simulink library "lib_LargeBuildingModel"  (R2026a)
settings: Solver=VariableStepAuto
libraries: WallSelector_lib x380, ExternalWall_lib x188, RoomWithAirVolume x140, fl_lib x139, RoomLevelControl_lib x1
(part 11 of 12)

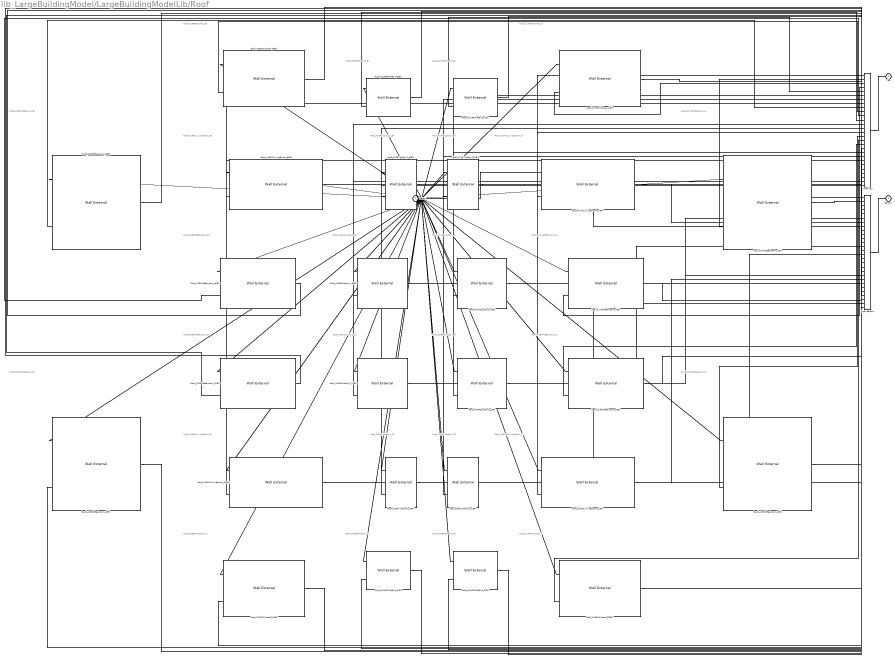
== system lib_LargeBuildingModel/LargeBuildingModelLib/Roof ==
  note: Roof_A17R1(LivingRoom_A)
  note: Roof_A17R2(Bedroom_A)
  note: Roof_A17R3(Kitchen_A)
  note: Roof_A17R4(Bathroom_A)
  note: Roof_A17R5(FireExit_A)
  note: Roof_A17R6(Lobby1_A)
  note: Roof_A17R7(Lobby2_A)
  note: Roof_A18R1(LivingRoom_B)
  note: Roof_A18R2(Bedroom_B)
  note: Roof_A18R3(Kitchen_B)
  note: Roof_A18R4(Bathroom_B)
  note: Roof_A18R5(FireExit_B)
  note: Roof_A18R6(Lobby1_B)
  note: Roof_A18R7(Lobby2_B)
  note: Roof_A19R1(LivingRoom_C)
  note: Roof_A19R2(Bedroom_C)
  note: Roof_A19R3(Kitchen_C)
  note: Roof_A19R4(Bathroom_C)
  note: Roof_A19R5(FireExit_C)
  note: Roof_A19R6(Lobby1_C)
  note: Roof_A19R7(Lobby2_C)
  note: Roof_A20R1(LivingRoom_D)
  note: Roof_A20R2(Bedroom_D)
  note: Roof_A20R3(Kitchen_D)
  note: Roof_A20R4(Bathroom_D)
  note: Roof_A20R5(FireExit_D)
  note: Roof_A20R6(Lobby1_D)
  note: Roof_A20R7(Lobby2_D)
  ArrayBottom : SimscapeArrayConnection  Domain=foundation.thermal.thermal  ConcatenateDimension=1  NumScalarElements=28
  ArrayTop : SimscapeArrayConnection  Domain=foundation.thermal.thermal  ConcatenateDimension=1  NumScalarElements=28
  Roof_A17R1(LivingRoom_A)Blk : ExternalWall_lib/Wall External  extWallModel=wallExternalModelOption.wallSolar  wallLength=2.4384 % Parameterized on : 13-Jun-2026 10:47:16 m  wallHeight=4.572 % Parameterized on : 13-Jun-2026 10:47:16 m  wallThickness=0.03 % Parameterized on : 13-Jun-2026 10:47:16 m  wallMaterialDen=1400 % Parameterized on : 13-Jun-2026 10:47:30 kg/m^3  wallMaterialCp=1000 % Parameterized on : 13-Jun-2026 10:47:30 J/(K*kg)  wallAbsorptivity=0.5  wallThermalK=0.7 % Parameterized on : 13-Jun-2026 10:47:30 W/(K*m)  winLength=1 m  winHeight=0.5 m  winThickness=0.007 m  winMaterialDen=2500 kg/m^3  winMaterialCp=787 J/(K*kg)  winAbsorptivity=0.35  winThermalK=1 W/(K*m)  winTransmissivity=0.45  ventLength=0.1 m  ventHeight=0.1 m  extToWallHTC=30 % Parameterized on : 13-Jun-2026 10:47:30 W/(K*m^2)  intToRoomHTC=30 % Parameterized on : 13-Jun-2026 10:47:30 W/(K*m^2)  iniT=300 % Parameterized on : 13-Jun-2026 10:47:30 K  latitude=5  longitude=5  localTime=5  dayLightS=0  surfAngle=90 deg  surfUnitV=[0, -1]  startYear=2025  startMonth=1  startDay=1  startHr=1  numHrsData=24  interp_method=simscape.enum.interpolation.linear  extrap_method=simscape.enum.extrapolation.nearest
  Roof_A17R2(Bedroom_A)Blk : ExternalWall_lib/Wall External  extWallModel=wallExternalModelOption.wallSolar  wallLength=4.2672 % Parameterized on : 13-Jun-2026 10:47:16 m  wallHeight=4.572 % Parameterized on : 13-Jun-2026 10:47:16 m  wallThickness=0.03 % Parameterized on : 13-Jun-2026 10:47:16 m  wallMaterialDen=1400 % Parameterized on : 13-Jun-2026 10:47:30 kg/m^3  wallMaterialCp=1000 % Parameterized on : 13-Jun-2026 10:47:30 J/(K*kg)  wallAbsorptivity=0.5  wallThermalK=0.7 % Parameterized on : 13-Jun-2026 10:47:30 W/(K*m)  winLength=1 m  winHeight=0.5 m  winThickness=0.007 m  winMaterialDen=2500 kg/m^3  winMaterialCp=787 J/(K*kg)  winAbsorptivity=0.35  winThermalK=1 W/(K*m)  winTransmissivity=0.45  ventLength=0.1 m  ventHeight=0.1 m  extToWallHTC=30 % Parameterized on : 13-Jun-2026 10:47:30 W/(K*m^2)  intToRoomHTC=30 % Parameterized on : 13-Jun-2026 10:47:30 W/(K*m^2)  iniT=300 % Parameterized on : 13-Jun-2026 10:47:30 K  latitude=5  longitude=5  localTime=5  dayLightS=0  surfAngle=90 deg  surfUnitV=[0, -1]  startYear=2025  startMonth=1  startDay=1  startHr=1  numHrsData=24  interp_method=simscape.enum.interpolation.linear  extrap_method=simscape.enum.extrapolation.nearest
  Roof_A17R3(Kitchen_A)Blk : ExternalWall_lib/Wall External  extWallModel=wallExternalModelOption.wallSolar  wallLength=2.7432 % Parameterized on : 13-Jun-2026 10:47:16 m  wallHeight=3.9624 % Parameterized on : 13-Jun-2026 10:47:16 m  wallThickness=0.03 % Parameterized on : 13-Jun-2026 10:47:16 m  wallMaterialDen=1400 % Parameterized on : 13-Jun-2026 10:47:30 kg/m^3  wallMaterialCp=1000 % Parameterized on : 13-Jun-2026 10:47:30 J/(K*kg)  wallAbsorptivity=0.5  wallThermalK=0.7 % Parameterized on : 13-Jun-2026 10:47:30 W/(K*m)  winLength=1 m  winHeight=0.5 m  winThickness=0.007 m  winMaterialDen=2500 kg/m^3  winMaterialCp=787 J/(K*kg)  winAbsorptivity=0.35  winThermalK=1 W/(K*m)  winTransmissivity=0.45  ventLength=0.1 m  ventHeight=0.1 m  extToWallHTC=30 % Parameterized on : 13-Jun-2026 10:47:30 W/(K*m^2)  intToRoomHTC=30 % Parameterized on : 13-Jun-2026 10:47:30 W/(K*m^2)  iniT=300 % Parameterized on : 13-Jun-2026 10:47:30 K  latitude=5  longitude=5  localTime=5  dayLightS=0  surfAngle=90 deg  surfUnitV=[0, -1]  startYear=2025  startMonth=1  startDay=1  startHr=1  numHrsData=24  interp_method=simscape.enum.interpolation.linear  extrap_method=simscape.enum.extrapolation.nearest
  Roof_A17R4(Bathroom_A)Blk : ExternalWall_lib/Wall External  extWallModel=wallExternalModelOption.wallSolar  wallLength=2.4384 % Parameterized on : 13-Jun-2026 10:47:16 m  wallHeight=3.6576 % Parameterized on : 13-Jun-2026 10:47:16 m  wallThickness=0.03 % Parameterized on : 13-Jun-2026 10:47:16 m  wallMaterialDen=1400 % Parameterized on : 13-Jun-2026 10:47:30 kg/m^3  wallMaterialCp=1000 % Parameterized on : 13-Jun-2026 10:47:30 J/(K*kg)  wallAbsorptivity=0.5  wallThermalK=0.7 % Parameterized on : 13-Jun-2026 10:47:30 W/(K*m)  winLength=1 m  winHeight=0.5 m  winThickness=0.007 m  winMaterialDen=2500 kg/m^3  winMaterialCp=787 J/(K*kg)  winAbsorptivity=0.35  winThermalK=1 W/(K*m)  winTransmissivity=0.45  ventLength=0.1 m  ventHeight=0.1 m  extToWallHTC=30 % Parameterized on : 13-Jun-2026 10:47:30 W/(K*m^2)  intToRoomHTC=30 % Parameterized on : 13-Jun-2026 10:47:30 W/(K*m^2)  iniT=300 % Parameterized on : 13-Jun-2026 10:47:30 K  latitude=5  longitude=5  localTime=5  dayLightS=0  surfAngle=90 deg  surfUnitV=[0, -1]  startYear=2025  startMonth=1  startDay=1  startHr=1  numHrsData=24  interp_method=simscape.enum.interpolation.linear  extrap_method=simscape.enum.extrapolation.nearest
  Roof_A17R5(FireExit_A)Blk : ExternalWall_lib/Wall External  extWallModel=wallExternalModelOption.wallSolar  wallLength=1.8288 % Parameterized on : 13-Jun-2026 10:47:16 m  wallHeight=2.1336 % Parameterized on : 13-Jun-2026 10:47:16 m  wallThickness=0.03 % Parameterized on : 13-Jun-2026 10:47:16 m  wallMaterialDen=1400 % Parameterized on : 13-Jun-2026 10:47:30 kg/m^3  wallMaterialCp=1000 % Parameterized on : 13-Jun-2026 10:47:30 J/(K*kg)  wallAbsorptivity=0.5  wallThermalK=0.7 % Parameterized on : 13-Jun-2026 10:47:30 W/(K*m)  winLength=1 m  winHeight=0.5 m  winThickness=0.007 m  winMaterialDen=2500 kg/m^3  winMaterialCp=787 J/(K*kg)  winAbsorptivity=0.35  winThermalK=1 W/(K*m)  winTransmissivity=0.45  ventLength=0.1 m  ventHeight=0.1 m  extToWallHTC=30 % Parameterized on : 13-Jun-2026 10:47:30 W/(K*m^2)  intToRoomHTC=30 % Parameterized on : 13-Jun-2026 10:47:30 W/(K*m^2)  iniT=300 % Parameterized on : 13-Jun-2026 10:47:30 K  latitude=5  longitude=5  localTime=5  dayLightS=0  surfAngle=90 deg  surfUnitV=[0, -1]  startYear=2025  startMonth=1  startDay=1  startHr=1  numHrsData=24  interp_method=simscape.enum.interpolation.linear  extrap_method=simscape.enum.extrapolation.nearest
  Roof_A17R6(Lobby1_A)Blk : ExternalWall_lib/Wall External  extWallModel=wallExternalModelOption.wallSolar  wallLength=2.4384 % Parameterized on : 13-Jun-2026 10:47:16 m  wallHeight=2.4384 % Parameterized on : 13-Jun-2026 10:47:16 m  wallThickness=0.03 % Parameterized on : 13-Jun-2026 10:47:16 m  wallMaterialDen=1400 % Parameterized on : 13-Jun-2026 10:47:30 kg/m^3  wallMaterialCp=1000 % Parameterized on : 13-Jun-2026 10:47:30 J/(K*kg)  wallAbsorptivity=0.5  wallThermalK=0.7 % Parameterized on : 13-Jun-2026 10:47:30 W/(K*m)  winLength=1 m  winHeight=0.5 m  winThickness=0.007 m  winMaterialDen=2500 kg/m^3  winMaterialCp=787 J/(K*kg)  winAbsorptivity=0.35  winThermalK=1 W/(K*m)  winTransmissivity=0.45  ventLength=0.1 m  ventHeight=0.1 m  extToWallHTC=30 % Parameterized on : 13-Jun-2026 10:47:30 W/(K*m^2)  intToRoomHTC=30 % Parameterized on : 13-Jun-2026 10:47:30 W/(K*m^2)  iniT=300 % Parameterized on : 13-Jun-2026 10:47:30 K  latitude=5  longitude=5  localTime=5  dayLightS=0  surfAngle=90 deg  surfUnitV=[0, -1]  startYear=2025  startMonth=1  startDay=1  startHr=1  numHrsData=24  interp_method=simscape.enum.interpolation.linear  extrap_method=simscape.enum.extrapolation.nearest
  Roof_A17R7(Lobby2_A)Blk : ExternalWall_lib/Wall External  extWallModel=wallExternalModelOption.wallSolar  wallLength=2.4384 % Parameterized on : 13-Jun-2026 10:47:16 m  wallHeight=1.524 % Parameterized on : 13-Jun-2026 10:47:16 m  wallThickness=0.03 % Parameterized on : 13-Jun-2026 10:47:16 m  wallMaterialDen=1400 % Parameterized on : 13-Jun-2026 10:47:30 kg/m^3  wallMaterialCp=1000 % Parameterized on : 13-Jun-2026 10:47:30 J/(K*kg)  wallAbsorptivity=0.5  wallThermalK=0.7 % Parameterized on : 13-Jun-2026 10:47:30 W/(K*m)  winLength=1 m  winHeight=0.5 m  winThickness=0.007 m  winMaterialDen=2500 kg/m^3  winMaterialCp=787 J/(K*kg)  winAbsorptivity=0.35  winThermalK=1 W/(K*m)  winTransmissivity=0.45  ventLength=0.1 m  ventHeight=0.1 m  extToWallHTC=30 % Parameterized on : 13-Jun-2026 10:47:30 W/(K*m^2)  intToRoomHTC=30 % Parameterized on : 13-Jun-2026 10:47:30 W/(K*m^2)  iniT=300 % Parameterized on : 13-Jun-2026 10:47:30 K  latitude=5  longitude=5  localTime=5  dayLightS=0  surfAngle=90 deg  surfUnitV=[0, -1]  startYear=2025  startMonth=1  startDay=1  startHr=1  numHrsData=24  interp_method=simscape.enum.interpolation.linear  extrap_method=simscape.enum.extrapolation.nearest
  Roof_A18R1(LivingRoom_B)Blk : ExternalWall_lib/Wall External  extWallModel=wallExternalModelOption.wallSolar  wallLength=2.4384 % Parameterized on : 13-Jun-2026 10:47:16 m  wallHeight=4.572 % Parameterized on : 13-Jun-2026 10:47:16 m  wallThickness=0.03 % Parameterized on : 13-Jun-2026 10:47:16 m  wallMaterialDen=1400 % Parameterized on : 13-Jun-2026 10:47:30 kg/m^3  wallMaterialCp=1000 % Parameterized on : 13-Jun-2026 10:47:30 J/(K*kg)  wallAbsorptivity=0.5  wallThermalK=0.7 % Parameterized on : 13-Jun-2026 10:47:30 W/(K*m)  winLength=1 m  winHeight=0.5 m  winThickness=0.007 m  winMaterialDen=2500 kg/m^3  winMaterialCp=787 J/(K*kg)  winAbsorptivity=0.35  winThermalK=1 W/(K*m)  winTransmissivity=0.45  ventLength=0.1 m  ventHeight=0.1 m  extToWallHTC=30 % Parameterized on : 13-Jun-2026 10:47:30 W/(K*m^2)  intToRoomHTC=30 % Parameterized on : 13-Jun-2026 10:47:30 W/(K*m^2)  iniT=300 % Parameterized on : 13-Jun-2026 10:47:30 K  latitude=5  longitude=5  localTime=5  dayLightS=0  surfAngle=90 deg  surfUnitV=[0, -1]  startYear=2025  startMonth=1  startDay=1  startHr=1  numHrsData=24  interp_method=simscape.enum.interpolation.linear  extrap_method=simscape.enum.extrapolation.nearest
  Roof_A18R2(Bedroom_B)Blk : ExternalWall_lib/Wall External  extWallModel=wallExternalModelOption.wallSolar  wallLength=4.2672 % Parameterized on : 13-Jun-2026 10:47:16 m  wallHeight=4.572 % Parameterized on : 13-Jun-2026 10:47:16 m  wallThickness=0.03 % Parameterized on : 13-Jun-2026 10:47:16 m  wallMaterialDen=1400 % Parameterized on : 13-Jun-2026 10:47:30 kg/m^3  wallMaterialCp=1000 % Parameterized on : 13-Jun-2026 10:47:31 J/(K*kg)  wallAbsorptivity=0.5  wallThermalK=0.7 % Parameterized on : 13-Jun-2026 10:47:31 W/(K*m)  winLength=1 m  winHeight=0.5 m  winThickness=0.007 m  winMaterialDen=2500 kg/m^3  winMaterialCp=787 J/(K*kg)  winAbsorptivity=0.35  winThermalK=1 W/(K*m)  winTransmissivity=0.45  ventLength=0.1 m  ventHeight=0.1 m  extToWallHTC=30 % Parameterized on : 13-Jun-2026 10:47:31 W/(K*m^2)  intToRoomHTC=30 % Parameterized on : 13-Jun-2026 10:47:31 W/(K*m^2)  iniT=300 % Parameterized on : 13-Jun-2026 10:47:31 K  latitude=5  longitude=5  localTime=5  dayLightS=0  surfAngle=90 deg  surfUnitV=[0, -1]  startYear=2025  startMonth=1  startDay=1  startHr=1  numHrsData=24  interp_method=simscape.enum.interpolation.linear  extrap_method=simscape.enum.extrapolation.nearest
  Roof_A18R3(Kitchen_B)Blk : ExternalWall_lib/Wall External  extWallModel=wallExternalModelOption.wallSolar  wallLength=2.7432 % Parameterized on : 13-Jun-2026 10:47:16 m  wallHeight=3.9624 % Parameterized on : 13-Jun-2026 10:47:16 m  wallThickness=0.03 % Parameterized on : 13-Jun-2026 10:47:16 m  wallMaterialDen=1400 % Parameterized on : 13-Jun-2026 10:47:31 kg/m^3  wallMaterialCp=1000 % Parameterized on : 13-Jun-2026 10:47:31 J/(K*kg)  wallAbsorptivity=0.5  wallThermalK=0.7 % Parameterized on : 13-Jun-2026 10:47:31 W/(K*m)  winLength=1 m  winHeight=0.5 m  winThickness=0.007 m  winMaterialDen=2500 kg/m^3  winMaterialCp=787 J/(K*kg)  winAbsorptivity=0.35  winThermalK=1 W/(K*m)  winTransmissivity=0.45  ventLength=0.1 m  ventHeight=0.1 m  extToWallHTC=30 % Parameterized on : 13-Jun-2026 10:47:31 W/(K*m^2)  intToRoomHTC=30 % Parameterized on : 13-Jun-2026 10:47:31 W/(K*m^2)  iniT=300 % Parameterized on : 13-Jun-2026 10:47:31 K  latitude=5  longitude=5  localTime=5  dayLightS=0  surfAngle=90 deg  surfUnitV=[0, -1]  startYear=2025  startMonth=1  startDay=1  startHr=1  numHrsData=24  interp_method=simscape.enum.interpolation.linear  extrap_method=simscape.enum.extrapolation.nearest
  Roof_A18R4(Bathroom_B)Blk : ExternalWall_lib/Wall External  extWallModel=wallExternalModelOption.wallSolar  wallLength=2.4384 % Parameterized on : 13-Jun-2026 10:47:16 m  wallHeight=3.6576 % Parameterized on : 13-Jun-2026 10:47:16 m  wallThickness=0.03 % Parameterized on : 13-Jun-2026 10:47:16 m  wallMaterialDen=1400 % Parameterized on : 13-Jun-2026 10:47:31 kg/m^3  wallMaterialCp=1000 % Parameterized on : 13-Jun-2026 10:47:31 J/(K*kg)  wallAbsorptivity=0.5  wallThermalK=0.7 % Parameterized on : 13-Jun-2026 10:47:31 W/(K*m)  winLength=1 m  winHeight=0.5 m  winThickness=0.007 m  winMaterialDen=2500 kg/m^3  winMaterialCp=787 J/(K*kg)  winAbsorptivity=0.35  winThermalK=1 W/(K*m)  winTransmissivity=0.45  ventLength=0.1 m  ventHeight=0.1 m  extToWallHTC=30 % Parameterized on : 13-Jun-2026 10:47:31 W/(K*m^2)  intToRoomHTC=30 % Parameterized on : 13-Jun-2026 10:47:31 W/(K*m^2)  iniT=300 % Parameterized on : 13-Jun-2026 10:47:31 K  latitude=5  longitude=5  localTime=5  dayLightS=0  surfAngle=90 deg  surfUnitV=[0, -1]  startYear=2025  startMonth=1  startDay=1  startHr=1  numHrsData=24  interp_method=simscape.enum.interpolation.linear  extrap_method=simscape.enum.extrapolation.nearest
  Roof_A18R5(FireExit_B)Blk : ExternalWall_lib/Wall External  extWallModel=wallExternalModelOption.wallSolar  wallLength=1.8288 % Parameterized on : 13-Jun-2026 10:47:16 m  wallHeight=2.1336 % Parameterized on : 13-Jun-2026 10:47:16 m  wallThickness=0.03 % Parameterized on : 13-Jun-2026 10:47:16 m  wallMaterialDen=1400 % Parameterized on : 13-Jun-2026 10:47:31 kg/m^3  wallMaterialCp=1000 % Parameterized on : 13-Jun-2026 10:47:31 J/(K*kg)  wallAbsorptivity=0.5  wallThermalK=0.7 % Parameterized on : 13-Jun-2026 10:47:31 W/(K*m)  winLength=1 m  winHeight=0.5 m  winThickness=0.007 m  winMaterialDen=2500 kg/m^3  winMaterialCp=787 J/(K*kg)  winAbsorptivity=0.35  winThermalK=1 W/(K*m)  winTransmissivity=0.45  ventLength=0.1 m  ventHeight=0.1 m  extToWallHTC=30 % Parameterized on : 13-Jun-2026 10:47:31 W/(K*m^2)  intToRoomHTC=30 % Parameterized on : 13-Jun-2026 10:47:31 W/(K*m^2)  iniT=300 % Parameterized on : 13-Jun-2026 10:47:31 K  latitude=5  longitude=5  localTime=5  dayLightS=0  surfAngle=90 deg  surfUnitV=[0, -1]  startYear=2025  startMonth=1  startDay=1  startHr=1  numHrsData=24  interp_method=simscape.enum.interpolation.linear  extrap_method=simscape.enum.extrapolation.nearest
  Roof_A18R6(Lobby1_B)Blk : ExternalWall_lib/Wall External  extWallModel=wallExternalModelOption.wallSolar  wallLength=2.4384 % Parameterized on : 13-Jun-2026 10:47:16 m  wallHeight=2.4384 % Parameterized on : 13-Jun-2026 10:47:16 m  wallThickness=0.03 % Parameterized on : 13-Jun-2026 10:47:16 m  wallMaterialDen=1400 % Parameterized on : 13-Jun-2026 10:47:31 kg/m^3  wallMaterialCp=1000 % Parameterized on : 13-Jun-2026 10:47:31 J/(K*kg)  wallAbsorptivity=0.5  wallThermalK=0.7 % Parameterized on : 13-Jun-2026 10:47:31 W/(K*m)  winLength=1 m  winHeight=0.5 m  winThickness=0.007 m  winMaterialDen=2500 kg/m^3  winMaterialCp=787 J/(K*kg)  winAbsorptivity=0.35  winThermalK=1 W/(K*m)  winTransmissivity=0.45  ventLength=0.1 m  ventHeight=0.1 m  extToWallHTC=30 % Parameterized on : 13-Jun-2026 10:47:31 W/(K*m^2)  intToRoomHTC=30 % Parameterized on : 13-Jun-2026 10:47:31 W/(K*m^2)  iniT=300 % Parameterized on : 13-Jun-2026 10:47:31 K  latitude=5  longitude=5  localTime=5  dayLightS=0  surfAngle=90 deg  surfUnitV=[0, -1]  startYear=2025  startMonth=1  startDay=1  startHr=1  numHrsData=24  interp_method=simscape.enum.interpolation.linear  extrap_method=simscape.enum.extrapolation.nearest
  Roof_A18R7(Lobby2_B)Blk : ExternalWall_lib/Wall External  extWallModel=wallExternalModelOption.wallSolar  wallLength=2.4384 % Parameterized on : 13-Jun-2026 10:47:16 m  wallHeight=1.524 % Parameterized on : 13-Jun-2026 10:47:16 m  wallThickness=0.03 % Parameterized on : 13-Jun-2026 10:47:16 m  wallMaterialDen=1400 % Parameterized on : 13-Jun-2026 10:47:31 kg/m^3  wallMaterialCp=1000 % Parameterized on : 13-Jun-2026 10:47:31 J/(K*kg)  wallAbsorptivity=0.5  wallThermalK=0.7 % Parameterized on : 13-Jun-2026 10:47:31 W/(K*m)  winLength=1 m  winHeight=0.5 m  winThickness=0.007 m  winMaterialDen=2500 kg/m^3  winMaterialCp=787 J/(K*kg)  winAbsorptivity=0.35  winThermalK=1 W/(K*m)  winTransmissivity=0.45  ventLength=0.1 m  ventHeight=0.1 m  extToWallHTC=30 % Parameterized on : 13-Jun-2026 10:47:31 W/(K*m^2)  intToRoomHTC=30 % Parameterized on : 13-Jun-2026 10:47:31 W/(K*m^2)  iniT=300 % Parameterized on : 13-Jun-2026 10:47:31 K  latitude=5  longitude=5  localTime=5  dayLightS=0  surfAngle=90 deg  surfUnitV=[0, -1]  startYear=2025  startMonth=1  startDay=1  startHr=1  numHrsData=24  interp_method=simscape.enum.interpolation.linear  extrap_method=simscape.enum.extrapolation.nearest
  Roof_A19R1(LivingRoom_C)Blk : ExternalWall_lib/Wall External  extWallModel=wallExternalModelOption.wallSolar  wallLength=2.4384 % Parameterized on : 13-Jun-2026 10:47:16 m  wallHeight=4.572 % Parameterized on : 13-Jun-2026 10:47:16 m  wallThickness=0.03 % Parameterized on : 13-Jun-2026 10:47:16 m  wallMaterialDen=1400 % Parameterized on : 13-Jun-2026 10:47:31 kg/m^3  wallMaterialCp=1000 % Parameterized on : 13-Jun-2026 10:47:31 J/(K*kg)  wallAbsorptivity=0.5  wallThermalK=0.7 % Parameterized on : 13-Jun-2026 10:47:31 W/(K*m)  winLength=1 m  winHeight=0.5 m  winThickness=0.007 m  winMaterialDen=2500 kg/m^3  winMaterialCp=787 J/(K*kg)  winAbsorptivity=0.35  winThermalK=1 W/(K*m)  winTransmissivity=0.45  ventLength=0.1 m  ventHeight=0.1 m  extToWallHTC=30 % Parameterized on : 13-Jun-2026 10:47:31 W/(K*m^2)  intToRoomHTC=30 % Parameterized on : 13-Jun-2026 10:47:31 W/(K*m^2)  iniT=300 % Parameterized on : 13-Jun-2026 10:47:31 K  latitude=5  longitude=5  localTime=5  dayLightS=0  surfAngle=90 deg  surfUnitV=[0, -1]  startYear=2025  startMonth=1  startDay=1  startHr=1  numHrsData=24  interp_method=simscape.enum.interpolation.linear  extrap_method=simscape.enum.extrapolation.nearest
  Roof_A19R2(Bedroom_C)Blk : ExternalWall_lib/Wall External  extWallModel=wallExternalModelOption.wallSolar  wallLength=4.2672 % Parameterized on : 13-Jun-2026 10:47:16 m  wallHeight=4.572 % Parameterized on : 13-Jun-2026 10:47:16 m  wallThickness=0.03 % Parameterized on : 13-Jun-2026 10:47:16 m  wallMaterialDen=1400 % Parameterized on : 13-Jun-2026 10:47:31 kg/m^3  wallMaterialCp=1000 % Parameterized on : 13-Jun-2026 10:47:31 J/(K*kg)  wallAbsorptivity=0.5  wallThermalK=0.7 % Parameterized on : 13-Jun-2026 10:47:31 W/(K*m)  winLength=1 m  winHeight=0.5 m  winThickness=0.007 m  winMaterialDen=2500 kg/m^3  winMaterialCp=787 J/(K*kg)  winAbsorptivity=0.35  winThermalK=1 W/(K*m)  winTransmissivity=0.45  ventLength=0.1 m  ventHeight=0.1 m  extToWallHTC=30 % Parameterized on : 13-Jun-2026 10:47:31 W/(K*m^2)  intToRoomHTC=30 % Parameterized on : 13-Jun-2026 10:47:31 W/(K*m^2)  iniT=300 % Parameterized on : 13-Jun-2026 10:47:31 K  latitude=5  longitude=5  localTime=5  dayLightS=0  surfAngle=90 deg  surfUnitV=[0, -1]  startYear=2025  startMonth=1  startDay=1  startHr=1  numHrsData=24  interp_method=simscape.enum.interpolation.linear  extrap_method=simscape.enum.extrapolation.nearest
  Roof_A19R3(Kitchen_C)Blk : ExternalWall_lib/Wall External  extWallModel=wallExternalModelOption.wallSolar  wallLength=2.7432 % Parameterized on : 13-Jun-2026 10:47:16 m  wallHeight=3.9624 % Parameterized on : 13-Jun-2026 10:47:16 m  wallThickness=0.03 % Parameterized on : 13-Jun-2026 10:47:16 m  wallMaterialDen=1400 % Parameterized on : 13-Jun-2026 10:47:31 kg/m^3  wallMaterialCp=1000 % Parameterized on : 13-Jun-2026 10:47:31 J/(K*kg)  wallAbsorptivity=0.5  wallThermalK=0.7 % Parameterized on : 13-Jun-2026 10:47:31 W/(K*m)  winLength=1 m  winHeight=0.5 m  winThickness=0.007 m  winMaterialDen=2500 kg/m^3  winMaterialCp=787 J/(K*kg)  winAbsorptivity=0.35  winThermalK=1 W/(K*m)  winTransmissivity=0.45  ventLength=0.1 m  ventHeight=0.1 m  extToWallHTC=30 % Parameterized on : 13-Jun-2026 10:47:31 W/(K*m^2)  intToRoomHTC=30 % Parameterized on : 13-Jun-2026 10:47:31 W/(K*m^2)  iniT=300 % Parameterized on : 13-Jun-2026 10:47:31 K  latitude=5  longitude=5  localTime=5  dayLightS=0  surfAngle=90 deg  surfUnitV=[0, -1]  startYear=2025  startMonth=1  startDay=1  startHr=1  numHrsData=24  interp_method=simscape.enum.interpolation.linear  extrap_method=simscape.enum.extrapolation.nearest
  Roof_A19R4(Bathroom_C)Blk : ExternalWall_lib/Wall External  extWallModel=wallExternalModelOption.wallSolar  wallLength=2.4384 % Parameterized on : 13-Jun-2026 10:47:16 m  wallHeight=3.6576 % Parameterized on : 13-Jun-2026 10:47:16 m  wallThickness=0.03 % Parameterized on : 13-Jun-2026 10:47:16 m  wallMaterialDen=1400 % Parameterized on : 13-Jun-2026 10:47:31 kg/m^3  wallMaterialCp=1000 % Parameterized on : 13-Jun-2026 10:47:31 J/(K*kg)  wallAbsorptivity=0.5  wallThermalK=0.7 % Parameterized on : 13-Jun-2026 10:47:31 W/(K*m)  winLength=1 m  winHeight=0.5 m  winThickness=0.007 m  winMaterialDen=2500 kg/m^3  winMaterialCp=787 J/(K*kg)  winAbsorptivity=0.35  winThermalK=1 W/(K*m)  winTransmissivity=0.45  ventLength=0.1 m  ventHeight=0.1 m  extToWallHTC=30 % Parameterized on : 13-Jun-2026 10:47:31 W/(K*m^2)  intToRoomHTC=30 % Parameterized on : 13-Jun-2026 10:47:31 W/(K*m^2)  iniT=300 % Parameterized on : 13-Jun-2026 10:47:31 K  latitude=5  longitude=5  localTime=5  dayLightS=0  surfAngle=90 deg  surfUnitV=[0, -1]  startYear=2025  startMonth=1  startDay=1  startHr=1  numHrsData=24  interp_method=simscape.enum.interpolation.linear  extrap_method=simscape.enum.extrapolation.nearest
  Roof_A19R5(FireExit_C)Blk : ExternalWall_lib/Wall External  extWallModel=wallExternalModelOption.wallSolar  wallLength=1.8288 % Parameterized on : 13-Jun-2026 10:47:16 m  wallHeight=2.1336 % Parameterized on : 13-Jun-2026 10:47:16 m  wallThickness=0.03 % Parameterized on : 13-Jun-2026 10:47:16 m  wallMaterialDen=1400 % Parameterized on : 13-Jun-2026 10:47:31 kg/m^3  wallMaterialCp=1000 % Parameterized on : 13-Jun-2026 10:47:31 J/(K*kg)  wallAbsorptivity=0.5  wallThermalK=0.7 % Parameterized on : 13-Jun-2026 10:47:31 W/(K*m)  winLength=1 m  winHeight=0.5 m  winThickness=0.007 m  winMaterialDen=2500 kg/m^3  winMaterialCp=787 J/(K*kg)  winAbsorptivity=0.35  winThermalK=1 W/(K*m)  winTransmissivity=0.45  ventLength=0.1 m  ventHeight=0.1 m  extToWallHTC=30 % Parameterized on : 13-Jun-2026 10:47:31 W/(K*m^2)  intToRoomHTC=30 % Parameterized on : 13-Jun-2026 10:47:31 W/(K*m^2)  iniT=300 % Parameterized on : 13-Jun-2026 10:47:31 K  latitude=5  longitude=5  localTime=5  dayLightS=0  surfAngle=90 deg  surfUnitV=[0, -1]  startYear=2025  startMonth=1  startDay=1  startHr=1  numHrsData=24  interp_method=simscape.enum.interpolation.linear  extrap_method=simscape.enum.extrapolation.nearest
  Roof_A19R6(Lobby1_C)Blk : ExternalWall_lib/Wall External  extWallModel=wallExternalModelOption.wallSolar  wallLength=2.4384 % Parameterized on : 13-Jun-2026 10:47:16 m  wallHeight=2.4384 % Parameterized on : 13-Jun-2026 10:47:16 m  wallThickness=0.03 % Parameterized on : 13-Jun-2026 10:47:16 m  wallMaterialDen=1400 % Parameterized on : 13-Jun-2026 10:47:31 kg/m^3  wallMaterialCp=1000 % Parameterized on : 13-Jun-2026 10:47:31 J/(K*kg)  wallAbsorptivity=0.5  wallThermalK=0.7 % Parameterized on : 13-Jun-2026 10:47:31 W/(K*m)  winLength=1 m  winHeight=0.5 m  winThickness=0.007 m  winMaterialDen=2500 kg/m^3  winMaterialCp=787 J/(K*kg)  winAbsorptivity=0.35  winThermalK=1 W/(K*m)  winTransmissivity=0.45  ventLength=0.1 m  ventHeight=0.1 m  extToWallHTC=30 % Parameterized on : 13-Jun-2026 10:47:31 W/(K*m^2)  intToRoomHTC=30 % Parameterized on : 13-Jun-2026 10:47:31 W/(K*m^2)  iniT=300 % Parameterized on : 13-Jun-2026 10:47:31 K  latitude=5  longitude=5  localTime=5  dayLightS=0  surfAngle=90 deg  surfUnitV=[0, -1]  startYear=2025  startMonth=1  startDay=1  startHr=1  numHrsData=24  interp_method=simscape.enum.interpolation.linear  extrap_method=simscape.enum.extrapolation.nearest
  Roof_A19R7(Lobby2_C)Blk : ExternalWall_lib/Wall External  extWallModel=wallExternalModelOption.wallSolar  wallLength=2.4384 % Parameterized on : 13-Jun-2026 10:47:16 m  wallHeight=1.524 % Parameterized on : 13-Jun-2026 10:47:16 m  wallThickness=0.03 % Parameterized on : 13-Jun-2026 10:47:16 m  wallMaterialDen=1400 % Parameterized on : 13-Jun-2026 10:47:31 kg/m^3  wallMaterialCp=1000 % Parameterized on : 13-Jun-2026 10:47:31 J/(K*kg)  wallAbsorptivity=0.5  wallThermalK=0.7 % Parameterized on : 13-Jun-2026 10:47:31 W/(K*m)  winLength=1 m  winHeight=0.5 m  winThickness=0.007 m  winMaterialDen=2500 kg/m^3  winMaterialCp=787 J/(K*kg)  winAbsorptivity=0.35  winThermalK=1 W/(K*m)  winTransmissivity=0.45  ventLength=0.1 m  ventHeight=0.1 m  extToWallHTC=30 % Parameterized on : 13-Jun-2026 10:47:31 W/(K*m^2)  intToRoomHTC=30 % Parameterized on : 13-Jun-2026 10:47:31 W/(K*m^2)  iniT=300 % Parameterized on : 13-Jun-2026 10:47:31 K  latitude=5  longitude=5  localTime=5  dayLightS=0  surfAngle=90 deg  surfUnitV=[0, -1]  startYear=2025  startMonth=1  startDay=1  startHr=1  numHrsData=24  interp_method=simscape.enum.interpolation.linear  extrap_method=simscape.enum.extrapolation.nearest
  Roof_A20R1(LivingRoom_D)Blk : ExternalWall_lib/Wall External  extWallModel=wallExternalModelOption.wallSolar  wallLength=2.4384 % Parameterized on : 13-Jun-2026 10:47:16 m  wallHeight=4.572 % Parameterized on : 13-Jun-2026 10:47:16 m  wallThickness=0.04 % Parameterized on : 13-Jun-2026 10:47:16 m  wallMaterialDen=2000 % Parameterized on : 13-Jun-2026 10:47:31 kg/m^3  wallMaterialCp=1100 % Parameterized on : 13-Jun-2026 10:47:31 J/(K*kg)  wallAbsorptivity=0.6 % Parameterized on : 13-Jun-2026 10:47:31  wallThermalK=1.4 % Parameterized on : 13-Jun-2026 10:47:31 W/(K*m)  winLength=1 m  winHeight=0.5 m  winThickness=0.007 m  winMaterialDen=2500 kg/m^3  winMaterialCp=787 J/(K*kg)  winAbsorptivity=0.35  winThermalK=1 W/(K*m)  winTransmissivity=0.45  ventLength=0.1 m  ventHeight=0.1 m  extToWallHTC=20 % Parameterized on : 13-Jun-2026 10:47:31 W/(K*m^2)  intToRoomHTC=30 % Parameterized on : 13-Jun-2026 10:47:31 W/(K*m^2)  iniT=300 % Parameterized on : 13-Jun-2026 10:47:31 K  latitude=5  longitude=5  localTime=5  dayLightS=0  surfAngle=0 % Parameterized on : 13-Jun-2026 10:47:16 deg  surfUnitV=[0,-1] % Parameterized on : 13-Jun-2026 10:47:16  startYear=2025  startMonth=1  startDay=1  startHr=1  numHrsData=24  interp_method=simscape.enum.interpolation.linear  extrap_method=simscape.enum.extrapolation.nearest
  Roof_A20R2(Bedroom_D)Blk : ExternalWall_lib/Wall External  extWallModel=wallExternalModelOption.wallSolar  wallLength=4.2672 % Parameterized on : 13-Jun-2026 10:47:16 m  wallHeight=4.572 % Parameterized on : 13-Jun-2026 10:47:16 m  wallThickness=0.04 % Parameterized on : 13-Jun-2026 10:47:16 m  wallMaterialDen=2000 % Parameterized on : 13-Jun-2026 10:47:31 kg/m^3  wallMaterialCp=1100 % Parameterized on : 13-Jun-2026 10:47:31 J/(K*kg)  wallAbsorptivity=0.6 % Parameterized on : 13-Jun-2026 10:47:31  wallThermalK=1.4 % Parameterized on : 13-Jun-2026 10:47:31 W/(K*m)  winLength=1 m  winHeight=0.5 m  winThickness=0.007 m  winMaterialDen=2500 kg/m^3  winMaterialCp=787 J/(K*kg)  winAbsorptivity=0.35  winThermalK=1 W/(K*m)  winTransmissivity=0.45  ventLength=0.1 m  ventHeight=0.1 m  extToWallHTC=20 % Parameterized on : 13-Jun-2026 10:47:31 W/(K*m^2)  intToRoomHTC=30 % Parameterized on : 13-Jun-2026 10:47:31 W/(K*m^2)  iniT=300 % Parameterized on : 13-Jun-2026 10:47:31 K  latitude=5  longitude=5  localTime=5  dayLightS=0  surfAngle=0 % Parameterized on : 13-Jun-2026 10:47:16 deg  surfUnitV=[0,-1] % Parameterized on : 13-Jun-2026 10:47:16  startYear=2025  startMonth=1  startDay=1  startHr=1  numHrsData=24  interp_method=simscape.enum.interpolation.linear  extrap_method=simscape.enum.extrapolation.nearest
  Roof_A20R3(Kitchen_D)Blk : ExternalWall_lib/Wall External  extWallModel=wallExternalModelOption.wallSolar  wallLength=2.7432 % Parameterized on : 13-Jun-2026 10:47:16 m  wallHeight=3.9624 % Parameterized on : 13-Jun-2026 10:47:16 m  wallThickness=0.04 % Parameterized on : 13-Jun-2026 10:47:16 m  wallMaterialDen=2000 % Parameterized on : 13-Jun-2026 10:47:31 kg/m^3  wallMaterialCp=1100 % Parameterized on : 13-Jun-2026 10:47:31 J/(K*kg)  wallAbsorptivity=0.6 % Parameterized on : 13-Jun-2026 10:47:31  wallThermalK=1.4 % Parameterized on : 13-Jun-2026 10:47:31 W/(K*m)  winLength=1 m  winHeight=0.5 m  winThickness=0.007 m  winMaterialDen=2500 kg/m^3  winMaterialCp=787 J/(K*kg)  winAbsorptivity=0.35  winThermalK=1 W/(K*m)  winTransmissivity=0.45  ventLength=0.1 m  ventHeight=0.1 m  extToWallHTC=20 % Parameterized on : 13-Jun-2026 10:47:31 W/(K*m^2)  intToRoomHTC=30 % Parameterized on : 13-Jun-2026 10:47:31 W/(K*m^2)  iniT=300 % Parameterized on : 13-Jun-2026 10:47:31 K  latitude=5  longitude=5  localTime=5  dayLightS=0  surfAngle=0 % Parameterized on : 13-Jun-2026 10:47:16 deg  surfUnitV=[0,-1] % Parameterized on : 13-Jun-2026 10:47:16  startYear=2025  startMonth=1  startDay=1  startHr=1  numHrsData=24  interp_method=simscape.enum.interpolation.linear  extrap_method=simscape.enum.extrapolation.nearest
  Roof_A20R4(Bathroom_D)Blk : ExternalWall_lib/Wall External  extWallModel=wallExternalModelOption.wallSolar  wallLength=2.4384 % Parameterized on : 13-Jun-2026 10:47:16 m  wallHeight=3.6576 % Parameterized on : 13-Jun-2026 10:47:16 m  wallThickness=0.04 % Parameterized on : 13-Jun-2026 10:47:16 m  wallMaterialDen=2000 % Parameterized on : 13-Jun-2026 10:47:31 kg/m^3  wallMaterialCp=1100 % Parameterized on : 13-Jun-2026 10:47:31 J/(K*kg)  wallAbsorptivity=0.6 % Parameterized on : 13-Jun-2026 10:47:31  wallThermalK=1.4 % Parameterized on : 13-Jun-2026 10:47:31 W/(K*m)  winLength=1 m  winHeight=0.5 m  winThickness=0.007 m  winMaterialDen=2500 kg/m^3  winMaterialCp=787 J/(K*kg)  winAbsorptivity=0.35  winThermalK=1 W/(K*m)  winTransmissivity=0.45  ventLength=0.1 m  ventHeight=0.1 m  extToWallHTC=20 % Parameterized on : 13-Jun-2026 10:47:31 W/(K*m^2)  intToRoomHTC=30 % Parameterized on : 13-Jun-2026 10:47:31 W/(K*m^2)  iniT=300 % Parameterized on : 13-Jun-2026 10:47:31 K  latitude=5  longitude=5  localTime=5  dayLightS=0  surfAngle=0 % Parameterized on : 13-Jun-2026 10:47:16 deg  surfUnitV=[0,-1] % Parameterized on : 13-Jun-2026 10:47:16  startYear=2025  startMonth=1  startDay=1  startHr=1  numHrsData=24  interp_method=simscape.enum.interpolation.linear  extrap_method=simscape.enum.extrapolation.nearest
  Roof_A20R5(FireExit_D)Blk : ExternalWall_lib/Wall External  extWallModel=wallExternalModelOption.wallSolar  wallLength=1.8288 % Parameterized on : 13-Jun-2026 10:47:16 m  wallHeight=2.1336 % Parameterized on : 13-Jun-2026 10:47:16 m  wallThickness=0.04 % Parameterized on : 13-Jun-2026 10:47:16 m  wallMaterialDen=2000 % Parameterized on : 13-Jun-2026 10:47:31 kg/m^3  wallMaterialCp=1100 % Parameterized on : 13-Jun-2026 10:47:31 J/(K*kg)  wallAbsorptivity=0.6 % Parameterized on : 13-Jun-2026 10:47:31  wallThermalK=1.4 % Parameterized on : 13-Jun-2026 10:47:31 W/(K*m)  winLength=1 m  winHeight=0.5 m  winThickness=0.007 m  winMaterialDen=2500 kg/m^3  winMaterialCp=787 J/(K*kg)  winAbsorptivity=0.35  winThermalK=1 W/(K*m)  winTransmissivity=0.45  ventLength=0.1 m  ventHeight=0.1 m  extToWallHTC=20 % Parameterized on : 13-Jun-2026 10:47:31 W/(K*m^2)  intToRoomHTC=30 % Parameterized on : 13-Jun-2026 10:47:31 W/(K*m^2)  iniT=300 % Parameterized on : 13-Jun-2026 10:47:31 K  latitude=5  longitude=5  localTime=5  dayLightS=0  surfAngle=0 % Parameterized on : 13-Jun-2026 10:47:16 deg  surfUnitV=[0,-1] % Parameterized on : 13-Jun-2026 10:47:16  startYear=2025  startMonth=1  startDay=1  startHr=1  numHrsData=24  interp_method=simscape.enum.interpolation.linear  extrap_method=simscape.enum.extrapolation.nearest
  Roof_A20R6(Lobby1_D)Blk : ExternalWall_lib/Wall External  extWallModel=wallExternalModelOption.wallSolar  wallLength=2.4384 % Parameterized on : 13-Jun-2026 10:47:16 m  wallHeight=2.4384 % Parameterized on : 13-Jun-2026 10:47:16 m  wallThickness=0.04 % Parameterized on : 13-Jun-2026 10:47:16 m  wallMaterialDen=2000 % Parameterized on : 13-Jun-2026 10:47:31 kg/m^3  wallMaterialCp=1100 % Parameterized on : 13-Jun-2026 10:47:31 J/(K*kg)  wallAbsorptivity=0.6 % Parameterized on : 13-Jun-2026 10:47:31  wallThermalK=1.4 % Parameterized on : 13-Jun-2026 10:47:31 W/(K*m)  winLength=1 m  winHeight=0.5 m  winThickness=0.007 m  winMaterialDen=2500 kg/m^3  winMaterialCp=787 J/(K*kg)  winAbsorptivity=0.35  winThermalK=1 W/(K*m)  winTransmissivity=0.45  ventLength=0.1 m  ventHeight=0.1 m  extToWallHTC=20 % Parameterized on : 13-Jun-2026 10:47:31 W/(K*m^2)  intToRoomHTC=30 % Parameterized on : 13-Jun-2026 10:47:31 W/(K*m^2)  iniT=300 % Parameterized on : 13-Jun-2026 10:47:31 K  latitude=5  longitude=5  localTime=5  dayLightS=0  surfAngle=0 % Parameterized on : 13-Jun-2026 10:47:16 deg  surfUnitV=[0,-1] % Parameterized on : 13-Jun-2026 10:47:16  startYear=2025  startMonth=1  startDay=1  startHr=1  numHrsData=24  interp_method=simscape.enum.interpolation.linear  extrap_method=simscape.enum.extrapolation.nearest
  Roof_A20R7(Lobby2_D)Blk : ExternalWall_lib/Wall External  extWallModel=wallExternalModelOption.wallSolar  wallLength=2.4384 % Parameterized on : 13-Jun-2026 10:47:16 m  wallHeight=1.524 % Parameterized on : 13-Jun-2026 10:47:16 m  wallThickness=0.04 % Parameterized on : 13-Jun-2026 10:47:16 m  wallMaterialDen=2000 % Parameterized on : 13-Jun-2026 10:47:31 kg/m^3  wallMaterialCp=1100 % Parameterized on : 13-Jun-2026 10:47:31 J/(K*kg)  wallAbsorptivity=0.6 % Parameterized on : 13-Jun-2026 10:47:31  wallThermalK=1.4 % Parameterized on : 13-Jun-2026 10:47:31 W/(K*m)  winLength=1 m  winHeight=0.5 m  winThickness=0.007 m  winMaterialDen=2500 kg/m^3  winMaterialCp=787 J/(K*kg)  winAbsorptivity=0.35  winThermalK=1 W/(K*m)  winTransmissivity=0.45  ventLength=0.1 m  ventHeight=0.1 m  extToWallHTC=20 % Parameterized on : 13-Jun-2026 10:47:31 W/(K*m^2)  intToRoomHTC=30 % Parameterized on : 13-Jun-2026 10:47:31 W/(K*m^2)  iniT=300 % Parameterized on : 13-Jun-2026 10:47:31 K  latitude=5  longitude=5  localTime=5  dayLightS=0  surfAngle=0 % Parameterized on : 13-Jun-2026 10:47:16 deg  surfUnitV=[0,-1] % Parameterized on : 13-Jun-2026 10:47:16  startYear=2025  startMonth=1  startDay=1  startHr=1  numHrsData=24  interp_method=simscape.enum.interpolation.linear  extrap_method=simscape.enum.extrapolation.nearest
  Solar : PMIOPort  Side=Left
  Top : PMIOPort  Port=2  Side=Left
  Bottom : PMIOPort  Port=3  Side=Right
  connections:
  Roof_A17R1(LivingRoom_A)Blk/LConn1 -- Roof_A17R2(Bedroom_A)Blk/LConn1 -- Roof_A17R3(Kitchen_A)Blk/LConn1 -- Roof_A17R4(Bathroom_A)Blk/LConn1 -- Roof_A17R5(FireExit_A)Blk/LConn1 -- Roof_A17R6(Lobby1_A)Blk/LConn1 -- Roof_A17R7(Lobby2_A)Blk/LConn1 -- Roof_A18R1(LivingRoom_B)Blk/LConn1 -- Roof_A18R2(Bedroom_B)Blk/LConn1 -- Roof_A18R3(Kitchen_B)Blk/LConn1 -- Roof_A18R4(Bathroom_B)Blk/LConn1 -- Roof_A18R5(FireExit_B)Blk/LConn1 -- Roof_A18R6(Lobby1_B)Blk/LConn1 -- Roof_A18R7(Lobby2_B)Blk/LConn1 -- Roof_A19R1(LivingRoom_C)Blk/LConn1 -- Roof_A19R2(Bedroom_C)Blk/LConn1 -- Roof_A19R3(Kitchen_C)Blk/LConn1 -- Roof_A19R4(Bathroom_C)Blk/LConn1 -- Roof_A19R5(FireExit_C)Blk/LConn1 -- Roof_A19R6(Lobby1_C)Blk/LConn1 -- Roof_A19R7(Lobby2_C)Blk/LConn1 -- Roof_A20R1(LivingRoom_D)Blk/LConn1 -- Roof_A20R2(Bedroom_D)Blk/LConn1 -- Roof_A20R3(Kitchen_D)Blk/LConn1 -- Roof_A20R4(Bathroom_D)Blk/LConn1 -- Roof_A20R5(FireExit_D)Blk/LConn1 -- Roof_A20R6(Lobby1_D)Blk/LConn1 -- Solar/RConn1 -- Roof_A20R7(Lobby2_D)Blk/LConn1
  ArrayTop/RConn1 -- Top/RConn1
  Roof_A17R1(LivingRoom_A)Blk/LConn2 -- ArrayTop/LConn1
  Roof_A17R2(Bedroom_A)Blk/LConn2 -- ArrayTop/LConn2
  Roof_A17R3(Kitchen_A)Blk/LConn2 -- ArrayTop/LConn3
  Roof_A17R4(Bathroom_A)Blk/LConn2 -- ArrayTop/LConn4
  Roof_A17R5(FireExit_A)Blk/LConn2 -- ArrayTop/LConn5
  Roof_A17R6(Lobby1_A)Blk/LConn2 -- ArrayTop/LConn6
  Roof_A17R7(Lobby2_A)Blk/LConn2 -- ArrayTop/LConn7
  Roof_A18R1(LivingRoom_B)Blk/LConn2 -- ArrayTop/LConn8
  Roof_A18R2(Bedroom_B)Blk/LConn2 -- ArrayTop/LConn9
  Roof_A18R3(Kitchen_B)Blk/LConn2 -- ArrayTop/LConn10
  Roof_A18R4(Bathroom_B)Blk/LConn2 -- ArrayTop/LConn11
  Roof_A18R5(FireExit_B)Blk/LConn2 -- ArrayTop/LConn12
  Roof_A18R6(Lobby1_B)Blk/LConn2 -- ArrayTop/LConn13
  Roof_A18R7(Lobby2_B)Blk/LConn2 -- ArrayTop/LConn14
  Roof_A19R1(LivingRoom_C)Blk/LConn2 -- ArrayTop/LConn15
  Roof_A19R2(Bedroom_C)Blk/LConn2 -- ArrayTop/LConn16
  Roof_A19R3(Kitchen_C)Blk/LConn2 -- ArrayTop/LConn17
  Roof_A19R4(Bathroom_C)Blk/LConn2 -- ArrayTop/LConn18
  Roof_A19R5(FireExit_C)Blk/LConn2 -- ArrayTop/LConn19
  Roof_A19R6(Lobby1_C)Blk/LConn2 -- ArrayTop/LConn20
  Roof_A19R7(Lobby2_C)Blk/LConn2 -- ArrayTop/LConn21
  Roof_A20R1(LivingRoom_D)Blk/LConn2 -- ArrayTop/LConn22
  Roof_A20R2(Bedroom_D)Blk/LConn2 -- ArrayTop/LConn23
  Roof_A20R3(Kitchen_D)Blk/LConn2 -- ArrayTop/LConn24
  Roof_A20R4(Bathroom_D)Blk/LConn2 -- ArrayTop/LConn25
  Roof_A20R5(FireExit_D)Blk/LConn2 -- ArrayTop/LConn26
  Roof_A20R6(Lobby1_D)Blk/LConn2 -- ArrayTop/LConn27
  Roof_A20R7(Lobby2_D)Blk/LConn2 -- ArrayTop/LConn28
  ArrayBottom/RConn1 -- Bottom/RConn1
  Roof_A17R1(LivingRoom_A)Blk/RConn1 -- ArrayBottom/LConn1
  Roof_A17R2(Bedroom_A)Blk/RConn1 -- ArrayBottom/LConn2
  Roof_A17R3(Kitchen_A)Blk/RConn1 -- ArrayBottom/LConn3
  Roof_A17R4(Bathroom_A)Blk/RConn1 -- ArrayBottom/LConn4
  Roof_A17R5(FireExit_A)Blk/RConn1 -- ArrayBottom/LConn5
  Roof_A17R6(Lobby1_A)Blk/RConn1 -- ArrayBottom/LConn6
  Roof_A17R7(Lobby2_A)Blk/RConn1 -- ArrayBottom/LConn7
  Roof_A18R1(LivingRoom_B)Blk/RConn1 -- ArrayBottom/LConn8
  Roof_A18R2(Bedroom_B)Blk/RConn1 -- ArrayBottom/LConn9
  Roof_A18R3(Kitchen_B)Blk/RConn1 -- ArrayBottom/LConn10
  Roof_A18R4(Bathroom_B)Blk/RConn1 -- ArrayBottom/LConn11
  Roof_A18R5(FireExit_B)Blk/RConn1 -- ArrayBottom/LConn12
  Roof_A18R6(Lobby1_B)Blk/RConn1 -- ArrayBottom/LConn13
  Roof_A18R7(Lobby2_B)Blk/RConn1 -- ArrayBottom/LConn14
  Roof_A19R1(LivingRoom_C)Blk/RConn1 -- ArrayBottom/LConn15
  Roof_A19R2(Bedroom_C)Blk/RConn1 -- ArrayBottom/LConn16
  Roof_A19R3(Kitchen_C)Blk/RConn1 -- ArrayBottom/LConn17
  Roof_A19R4(Bathroom_C)Blk/RConn1 -- ArrayBottom/LConn18
  Roof_A19R5(FireExit_C)Blk/RConn1 -- ArrayBottom/LConn19
  Roof_A19R6(Lobby1_C)Blk/RConn1 -- ArrayBottom/LConn20
  Roof_A19R7(Lobby2_C)Blk/RConn1 -- ArrayBottom/LConn21
  Roof_A20R1(LivingRoom_D)Blk/RConn1 -- ArrayBottom/LConn22
  Roof_A20R2(Bedroom_D)Blk/RConn1 -- ArrayBottom/LConn23
  Roof_A20R3(Kitchen_D)Blk/RConn1 -- ArrayBottom/LConn24
  Roof_A20R4(Bathroom_D)Blk/RConn1 -- ArrayBottom/LConn25
  Roof_A20R5(FireExit_D)Blk/RConn1 -- ArrayBottom/LConn26
  Roof_A20R6(Lobby1_D)Blk/RConn1 -- ArrayBottom/LConn27
  Roof_A20R7(Lobby2_D)Blk/RConn1 -- ArrayBottom/LConn28

== system lib_LargeBuildingModel/LargeBuildingModelLib/roomT ==
  concat{1..4} (4 alike) : fl_lib/Physical Signals/Functions/PS Concatenate  catColumns=true
  1 : PMIOPort  Side=Left
  2 : PMIOPort  Port=2  Side=Left
  3 : PMIOPort  Port=3  Side=Left
  4 : PMIOPort  Port=4  Side=Left
  5 : PMIOPort  Port=5  Side=Left
  v : PMIOPort  Port=6  Side=Right
  connections:
  1/RConn1 -- concat1/LConn1
  2/RConn1 -- concat1/LConn2
  concat1/RConn1 -- concat2/LConn1
  3/RConn1 -- concat2/LConn2
  concat2/RConn1 -- concat3/LConn1
  4/RConn1 -- concat3/LConn2
  concat3/RConn1 -- concat4/LConn1
  5/RConn1 -- concat4/LConn2
  concat4/RConn1 -- v/RConn1

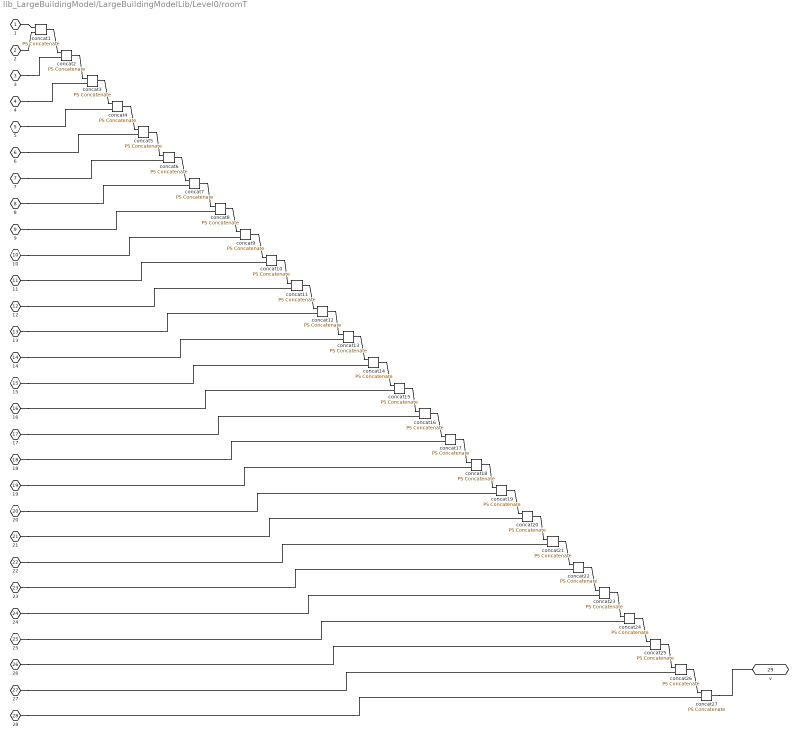
== system lib_LargeBuildingModel/LargeBuildingModelLib/Level0/roomT ==
  concat{1..27} (27 alike) : fl_lib/Physical Signals/Functions/PS Concatenate  catColumns=true
  1 : PMIOPort  Side=Left
  2 : PMIOPort  Port=2  Side=Left
  3 : PMIOPort  Port=3  Side=Left
  4 : PMIOPort  Port=4  Side=Left
  5 : PMIOPort  Port=5  Side=Left
  6 : PMIOPort  Port=6  Side=Left
  7 : PMIOPort  Port=7  Side=Left
  8 : PMIOPort  Port=8  Side=Left
  9 : PMIOPort  Port=9  Side=Left
  10 : PMIOPort  Port=10  Side=Left
  11 : PMIOPort  Port=11  Side=Left
  12 : PMIOPort  Port=12  Side=Left
  13 : PMIOPort  Port=13  Side=Left
  14 : PMIOPort  Port=14  Side=Left
  15 : PMIOPort  Port=15  Side=Left
  16 : PMIOPort  Port=16  Side=Left
  17 : PMIOPort  Port=17  Side=Left
  18 : PMIOPort  Port=18  Side=Left
  19 : PMIOPort  Port=19  Side=Left
  20 : PMIOPort  Port=20  Side=Left
  21 : PMIOPort  Port=21  Side=Left
  22 : PMIOPort  Port=22  Side=Left
  23 : PMIOPort  Port=23  Side=Left
  24 : PMIOPort  Port=24  Side=Left
  25 : PMIOPort  Port=25  Side=Left
  26 : PMIOPort  Port=26  Side=Left
  27 : PMIOPort  Port=27  Side=Left
  28 : PMIOPort  Port=28  Side=Left
  v : PMIOPort  Port=29  Side=Right
  connections:
  1/RConn1 -- concat1/LConn1
  2/RConn1 -- concat1/LConn2
  concat1/RConn1 -- concat2/LConn1
  3/RConn1 -- concat2/LConn2
  concat2/RConn1 -- concat3/LConn1
  4/RConn1 -- concat3/LConn2
  concat3/RConn1 -- concat4/LConn1
  5/RConn1 -- concat4/LConn2
  concat4/RConn1 -- concat5/LConn1
  6/RConn1 -- concat5/LConn2
  concat5/RConn1 -- concat6/LConn1
  7/RConn1 -- concat6/LConn2
  concat6/RConn1 -- concat7/LConn1
  8/RConn1 -- concat7/LConn2
  concat7/RConn1 -- concat8/LConn1
  9/RConn1 -- concat8/LConn2
  concat8/RConn1 -- concat9/LConn1
  10/RConn1 -- concat9/LConn2
  concat9/RConn1 -- concat10/LConn1
  11/RConn1 -- concat10/LConn2
  concat10/RConn1 -- concat11/LConn1
  12/RConn1 -- concat11/LConn2
  concat11/RConn1 -- concat12/LConn1
  13/RConn1 -- concat12/LConn2
  concat12/RConn1 -- concat13/LConn1
  14/RConn1 -- concat13/LConn2
  concat13/RConn1 -- concat14/LConn1
  15/RConn1 -- concat14/LConn2
  concat14/RConn1 -- concat15/LConn1
  16/RConn1 -- concat15/LConn2
  concat15/RConn1 -- concat16/LConn1
  17/RConn1 -- concat16/LConn2
  concat16/RConn1 -- concat17/LConn1
  18/RConn1 -- concat17/LConn2
  concat17/RConn1 -- concat18/LConn1
  19/RConn1 -- concat18/LConn2
  concat18/RConn1 -- concat19/LConn1
  20/RConn1 -- concat19/LConn2
  concat19/RConn1 -- concat20/LConn1
  21/RConn1 -- concat20/LConn2
  concat20/RConn1 -- concat21/LConn1
  22/RConn1 -- concat21/LConn2
  concat21/RConn1 -- concat22/LConn1
  23/RConn1 -- concat22/LConn2
  concat22/RConn1 -- concat23/LConn1
  24/RConn1 -- concat23/LConn2
  concat23/RConn1 -- concat24/LConn1
  25/RConn1 -- concat24/LConn2
  concat24/RConn1 -- concat25/LConn1
  26/RConn1 -- concat25/LConn2
  concat25/RConn1 -- concat26/LConn1
  27/RConn1 -- concat26/LConn2
  concat26/RConn1 -- concat27/LConn1
  28/RConn1 -- concat27/LConn2
  concat27/RConn1 -- v/RConn1

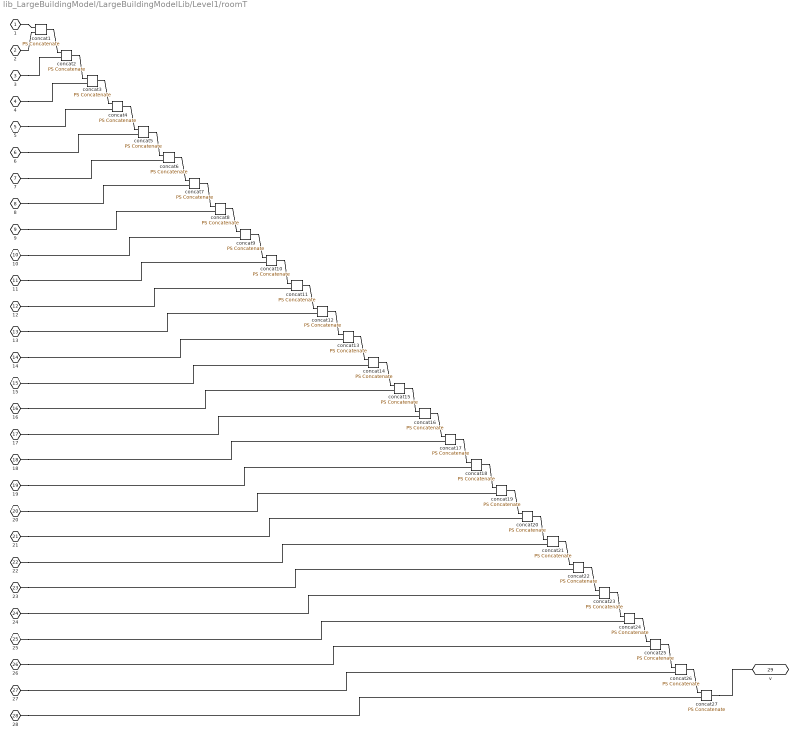
== system lib_LargeBuildingModel/LargeBuildingModelLib/Level1/roomT ==
  concat{1..27} (27 alike) : fl_lib/Physical Signals/Functions/PS Concatenate  catColumns=true
  1 : PMIOPort  Side=Left
  2 : PMIOPort  Port=2  Side=Left
  3 : PMIOPort  Port=3  Side=Left
  4 : PMIOPort  Port=4  Side=Left
  5 : PMIOPort  Port=5  Side=Left
  6 : PMIOPort  Port=6  Side=Left
  7 : PMIOPort  Port=7  Side=Left
  8 : PMIOPort  Port=8  Side=Left
  9 : PMIOPort  Port=9  Side=Left
  10 : PMIOPort  Port=10  Side=Left
  11 : PMIOPort  Port=11  Side=Left
  12 : PMIOPort  Port=12  Side=Left
  13 : PMIOPort  Port=13  Side=Left
  14 : PMIOPort  Port=14  Side=Left
  15 : PMIOPort  Port=15  Side=Left
  16 : PMIOPort  Port=16  Side=Left
  17 : PMIOPort  Port=17  Side=Left
  18 : PMIOPort  Port=18  Side=Left
  19 : PMIOPort  Port=19  Side=Left
  20 : PMIOPort  Port=20  Side=Left
  21 : PMIOPort  Port=21  Side=Left
  22 : PMIOPort  Port=22  Side=Left
  23 : PMIOPort  Port=23  Side=Left
  24 : PMIOPort  Port=24  Side=Left
  25 : PMIOPort  Port=25  Side=Left
  26 : PMIOPort  Port=26  Side=Left
  27 : PMIOPort  Port=27  Side=Left
  28 : PMIOPort  Port=28  Side=Left
  v : PMIOPort  Port=29  Side=Right
  connections:
  1/RConn1 -- concat1/LConn1
  2/RConn1 -- concat1/LConn2
  concat1/RConn1 -- concat2/LConn1
  3/RConn1 -- concat2/LConn2
  concat2/RConn1 -- concat3/LConn1
  4/RConn1 -- concat3/LConn2
  concat3/RConn1 -- concat4/LConn1
  5/RConn1 -- concat4/LConn2
  concat4/RConn1 -- concat5/LConn1
  6/RConn1 -- concat5/LConn2
  concat5/RConn1 -- concat6/LConn1
  7/RConn1 -- concat6/LConn2
  concat6/RConn1 -- concat7/LConn1
  8/RConn1 -- concat7/LConn2
  concat7/RConn1 -- concat8/LConn1
  9/RConn1 -- concat8/LConn2
  concat8/RConn1 -- concat9/LConn1
  10/RConn1 -- concat9/LConn2
  concat9/RConn1 -- concat10/LConn1
  11/RConn1 -- concat10/LConn2
  concat10/RConn1 -- concat11/LConn1
  12/RConn1 -- concat11/LConn2
  concat11/RConn1 -- concat12/LConn1
  13/RConn1 -- concat12/LConn2
  concat12/RConn1 -- concat13/LConn1
  14/RConn1 -- concat13/LConn2
  concat13/RConn1 -- concat14/LConn1
  15/RConn1 -- concat14/LConn2
  concat14/RConn1 -- concat15/LConn1
  16/RConn1 -- concat15/LConn2
  concat15/RConn1 -- concat16/LConn1
  17/RConn1 -- concat16/LConn2
  concat16/RConn1 -- concat17/LConn1
  18/RConn1 -- concat17/LConn2
  concat17/RConn1 -- concat18/LConn1
  19/RConn1 -- concat18/LConn2
  concat18/RConn1 -- concat19/LConn1
  20/RConn1 -- concat19/LConn2
  concat19/RConn1 -- concat20/LConn1
  21/RConn1 -- concat20/LConn2
  concat20/RConn1 -- concat21/LConn1
  22/RConn1 -- concat21/LConn2
  concat21/RConn1 -- concat22/LConn1
  23/RConn1 -- concat22/LConn2
  concat22/RConn1 -- concat23/LConn1
  24/RConn1 -- concat23/LConn2
  concat23/RConn1 -- concat24/LConn1
  25/RConn1 -- concat24/LConn2
  concat24/RConn1 -- concat25/LConn1
  26/RConn1 -- concat25/LConn2
  concat25/RConn1 -- concat26/LConn1
  27/RConn1 -- concat26/LConn2
  concat26/RConn1 -- concat27/LConn1
  28/RConn1 -- concat27/LConn2
  concat27/RConn1 -- v/RConn1
